simulink model "PT1_Filter_Demo"  (R2018a)
settings: Solver=FixedStepDiscrete  StartTime=0.0  StopTime=5  FixedStep=Ts_task  RelTol=1e-3
PreLoadFcn:
  | Ts_task = 0.001;
InitFcn:
  | if ~exist('Ts_task','var'), Ts_task = 0.001; end
settings Model: Creator=Ismail Shaikh  LastModifiedBy=Ismail Shaikh

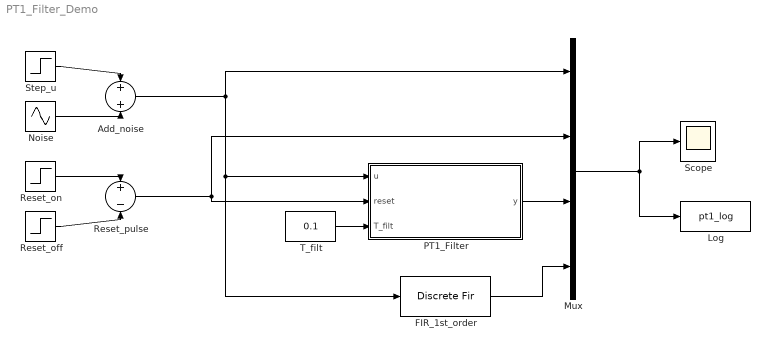
== system PT1_Filter_Demo ==
  Add_noise : Sum
  FIR_1st_order : DiscreteFir
  Log : ToWorkspace  VariableName=pt1_log  SaveFormat=Structure With Time  SampleTime=-1
  Mux : Mux
  Noise : Sin  Amplitude=0.2  Frequency=2*pi*50  SampleTime=Ts_task
  PT1_Filter : Subsystem  mask(PT1 Filter){Ts=Ts_task, y0=0}
      mask prompts: Ts "Task time Ts [s]"; y0 "Initial output y0"
      mask help: Discrete 1st-order low pass: y = y_prev + K*(u - y_prev), K = Ts/max(T_filt, Ts). reset~=0 sets y = u.
      mask Display: disp('PT1')
  Reset_off : Step  Time=3.05  SampleTime=Ts_task
  Reset_on : Step  Time=3  SampleTime=Ts_task
  Reset_pulse : Sum  Inputs=+-
  Scope : Scope
  Step_u : Step  Time=0.5  SampleTime=Ts_task
  T_filt : Constant  Value=0.1
  wires:
  Step_u/1 -> Add_noise/1
  Noise/1 -> Add_noise/2
  Reset_on/1 -> Reset_pulse/1
  Reset_off/1 -> Reset_pulse/2
  Add_noise/1 -> FIR_1st_order/1, PT1_Filter/1(u), Mux/1
  Reset_pulse/1 -> Mux/2, PT1_Filter/2(reset)
  T_filt/1 -> PT1_Filter/3(T_filt)
  PT1_Filter/1(y) -> Mux/3
  FIR_1st_order/1 -> Mux/4
  Mux/1 -> Scope/1, Log/1

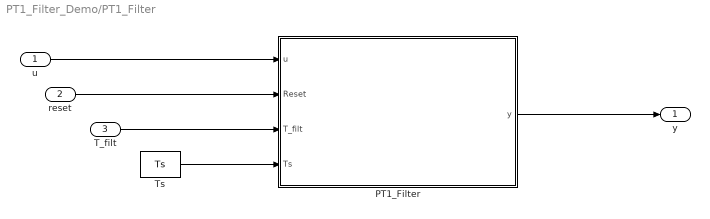
== system PT1_Filter_Demo/PT1_Filter ==
  u : Inport
  reset : Inport  Port=2
  T_filt : Inport  Port=3
  PT1_Filter : Subsystem
  Ts : Constant  Value=Ts
  y : Outport
  wires:
  u/1 -> PT1_Filter/1(u)
  reset/1 -> PT1_Filter/2(Reset)
  T_filt/1 -> PT1_Filter/3(T_filt)
  PT1_Filter/1(y) -> y/1
  Ts/1 -> PT1_Filter/4(Ts)

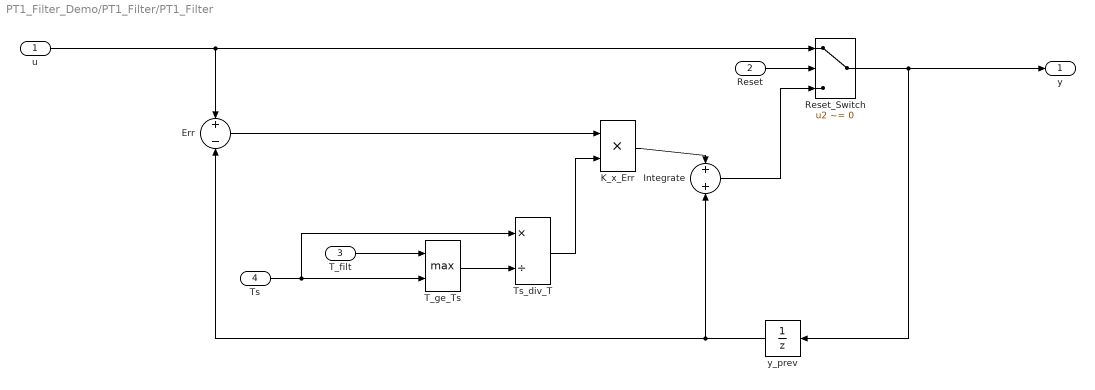
== system PT1_Filter_Demo/PT1_Filter/PT1_Filter ==
  u : Inport
  Reset : Inport  Port=2
  T_filt : Inport  Port=3
  Ts : Inport  Port=4
  Err : Sum  Inputs=+-
  Integrate : Sum
  K_x_Err : Product
  Reset_Switch : Switch  Criteria=u2 ~= 0
  T_ge_Ts : MinMax  Function=max  Inputs=2
  Ts_div_T : Product  Inputs=*/
  y_prev : UnitDelay  InitialCondition=y0  SampleTime=-1
  y : Outport
  wires:
  T_ge_Ts/1 -> Ts_div_T/2
  Err/1 -> K_x_Err/1
  u/1 -> Reset_Switch/1, Err/1
  Integrate/1 -> Reset_Switch/3
  Reset/1 -> Reset_Switch/2
  K_x_Err/1 -> Integrate/1
  y_prev/1 -> Err/2, Integrate/2
  T_filt/1 -> T_ge_Ts/1
  Ts_div_T/1 -> K_x_Err/2
  Reset_Switch/1 -> y_prev/1, y/1
  Ts/1 -> T_ge_Ts/2, Ts_div_T/1
